simulink model "scheme_L2"  (R2025b)
settings: Solver=VariableStepAuto  StartTime=0.0  StopTime=10.0  RelTol=1e-3
settings Model: Creator=yzhar  LastModifiedBy=user

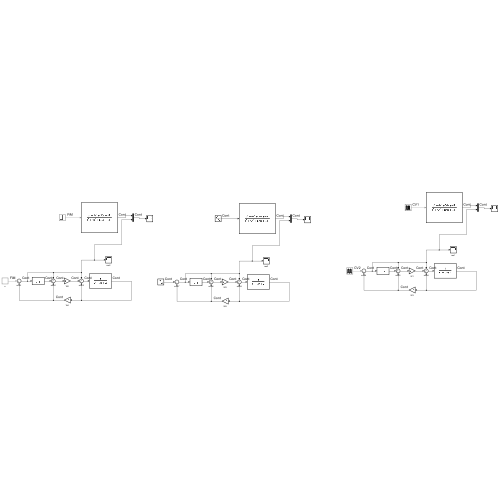
[thumbnail: Simulink's stored preview of the top-level diagram]
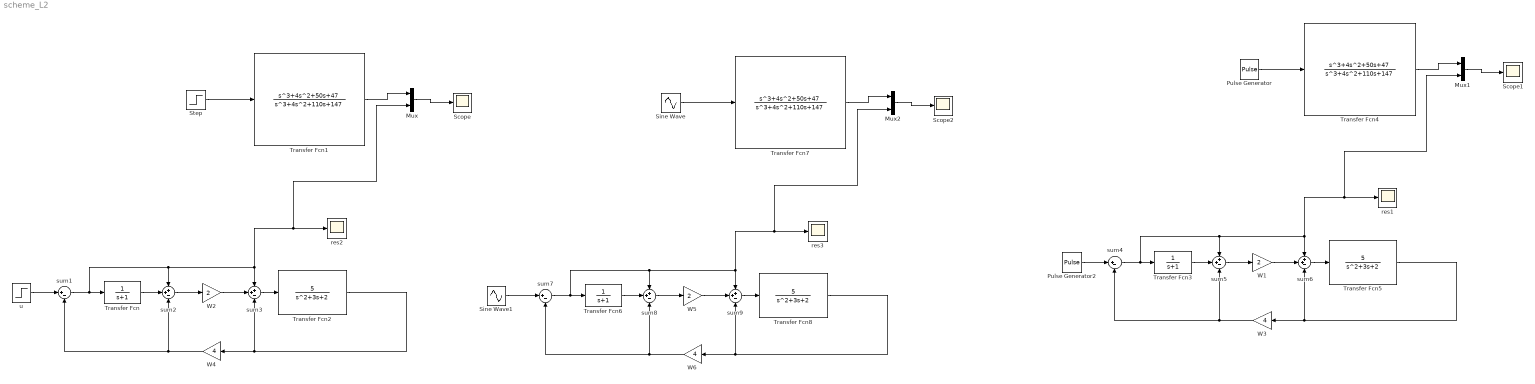
== system scheme_L2 ==
  Mux : Mux  Inputs=2
  Mux1 : Mux  Inputs=2
  Mux2 : Mux  Inputs=2
  Pulse Generator : DiscretePulseGenerator  PulseType=Time based  Period=100
  Pulse Generator2 : DiscretePulseGenerator  PulseType=Time based  Period=100
  Scope : Scope
      settings: ActiveDisplayYMinimum=-1  ActiveDisplayYMaximum=1
  Scope1 : Scope
      settings: ActiveDisplayYMinimum=-0.99391739859720152  ActiveDisplayYMaximum=1.2215463776219113  DataLoggingVariableName=ScopeData2
  Scope2 : Scope
      settings: ActiveDisplayYMinimum=-0.453027902214735  ActiveDisplayYMaximum=0.45383046996069132  DataLoggingVariableName=ScopeData4
  Sine Wave : Sin  SampleTime=0
  Sine Wave1 : Sin  SampleTime=0
  Step : Step  SampleTime=0
  Transfer Fcn : TransferFcn  Denominator=[1 1]
  Transfer Fcn1 : TransferFcn  Numerator=[1 4 50 47]  Denominator=[1 4 110 147]
  Transfer Fcn2 : TransferFcn  Numerator=[5]  Denominator=[1 3 2]
  Transfer Fcn3 : TransferFcn  Denominator=[1 1]
  Transfer Fcn4 : TransferFcn  Numerator=[1 4 50 47]  Denominator=[1 4 110 147]
  Transfer Fcn5 : TransferFcn  Numerator=[5]  Denominator=[1 3 2]
  Transfer Fcn6 : TransferFcn  Denominator=[1 1]
  Transfer Fcn7 : TransferFcn  Numerator=[1 4 50 47]  Denominator=[1 4 110 147]
  Transfer Fcn8 : TransferFcn  Numerator=[5]  Denominator=[1 3 2]
  W1 : Gain  Gain=2
  W2 : Gain  Gain=2
  W3 : Gain  Gain=4
  W4 : Gain  Gain=4
  W5 : Gain  Gain=2
  W6 : Gain  Gain=4
  res1 : Scope
      settings: ActiveDisplayYMinimum=-1.2863751525491946E+42  ActiveDisplayYMaximum=3.6595201315527205E+42  DataLoggingVariableName=ScopeData3
  res2 : Scope
      settings: ActiveDisplayYMinimum=-1.2863751525491946E+42  ActiveDisplayYMaximum=3.6595201315527205E+42
  res3 : Scope
      settings: ActiveDisplayYMinimum=-1.2863751525491946E+42  ActiveDisplayYMaximum=3.6595201315527205E+42  DataLoggingVariableName=ScopeData5
  sum1 : Sum  Inputs=|+-
  sum{2..3,5..6,8..9} (6 alike) : Sum  Inputs=++-
  sum4 : Sum  Inputs=|+-
  sum7 : Sum  Inputs=|+-
  u : Step  SampleTime=0
  wires:
  u/1 -> sum1/1
  sum1/1 -> Transfer Fcn/1, Mux/2, res2/1, sum3/1, sum2/1
  sum2/1 -> W2/1
  W2/1 -> sum3/2
  W4/1 -> sum1/2, sum2/3
  Transfer Fcn2/1 -> sum3/3, W4/1
  Transfer Fcn/1 -> sum2/2
  sum3/1 -> Transfer Fcn2/1
  Step/1 -> Transfer Fcn1/1
  Transfer Fcn1/1 -> Mux/1
  Mux/1 -> Scope/1
  Mux1/1 -> Scope1/1
  Transfer Fcn5/1 -> sum6/3, W3/1
  Transfer Fcn4/1 -> Mux1/1
  Transfer Fcn3/1 -> sum5/2
  sum6/1 -> Transfer Fcn5/1
  W3/1 -> sum4/2, sum5/3
  Pulse Generator2/1 -> sum4/1
  sum4/1 -> Transfer Fcn3/1, Mux1/2, res1/1, sum6/1, sum5/1
  sum5/1 -> W1/1
  W1/1 -> sum6/2
  Pulse Generator/1 -> Transfer Fcn4/1
  Mux2/1 -> Scope2/1
  Transfer Fcn8/1 -> sum9/3, W6/1
  Transfer Fcn7/1 -> Mux2/1
  Transfer Fcn6/1 -> sum8/2
  sum9/1 -> Transfer Fcn8/1
  W6/1 -> sum7/2, sum8/3
  sum7/1 -> Transfer Fcn6/1, Mux2/2, res3/1, sum9/1, sum8/1
  sum8/1 -> W5/1
  W5/1 -> sum9/2
  Sine Wave/1 -> Transfer Fcn7/1
  Sine Wave1/1 -> sum7/1
